simulink model "rc_sbus_encoder"  (R2026b)
settings: Solver=VariableStepAuto
undefined symbols (not defined in the file or in its folder): P, Ts
libraries: simulink x4
settings Model: Creator=aomar  LastModifiedBy=aomar

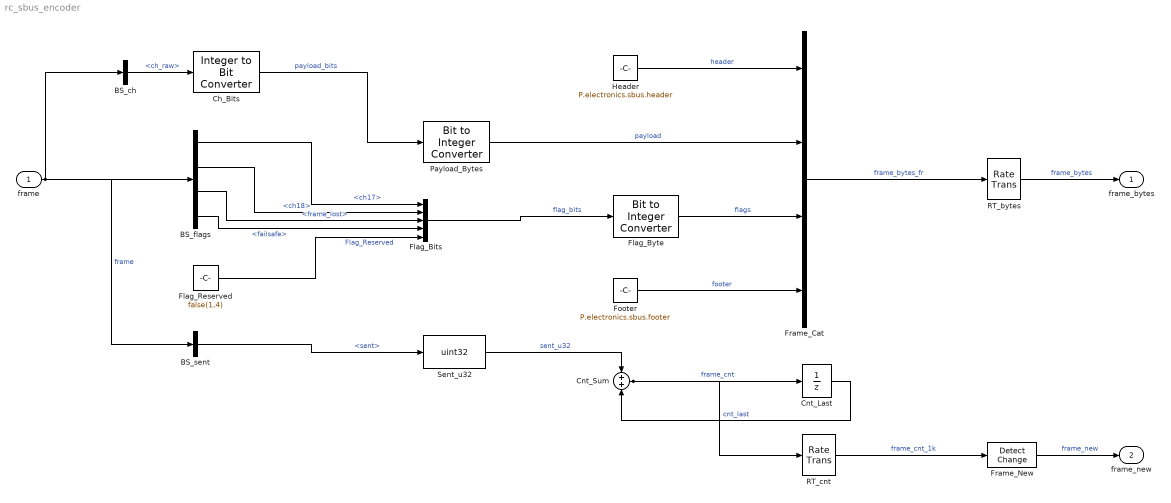
== system rc_sbus_encoder ==
  frame : Inport  OutDataTypeStr=Bus: Bus_RcFrame  SampleTime=Ts.rc_frame
  BS_ch : BusSelector  OutputSignals=ch_raw
  BS_flags : BusSelector  OutputSignals=ch17,ch18,frame_lost,failsafe
  BS_sent : BusSelector  OutputSignals=sent
  Ch_Bits : simulink/Logic and Bit Operations/Integer to Bit Converter  nbits=P.electronics.sbus.ch_bits  signedInputValues=Unsigned  bitOrder=LSB first  outDtype=boolean
      settings: LibrarySourceBlock=|
      | commutil2/Integer to Bit
      | Converter
  Cnt_Last : UnitDelay  SampleTime=Ts.rc_frame
  Cnt_Sum : Sum  OutDataTypeStr=uint32
  Flag_Bits : Concatenate  NumInputs=5
  Flag_Byte : simulink/Logic and Bit Operations/Bit to Integer Converter  nbits=8  bitOrder=LSB first  signedOutputValues=Unsigned  outDtype=uint8  outDtypeSigned=Inherit via internal rule
      settings: LibrarySourceBlock=|
      | commutil2/Bit to Integer
      | Converter
  Flag_Reserved : Constant  Value=false(1,4)  OutDataTypeStr=boolean  SampleTime=Ts.rc_frame
  Footer : Constant  Value=P.electronics.sbus.footer  OutDataTypeStr=uint8  SampleTime=Ts.rc_frame
  Frame_Cat : Concatenate  NumInputs=4
  Frame_New : simulink/Logic and Bit Operations/Detect Change  vinit=0  OutDataTypeStr=boolean
  Header : Constant  Value=P.electronics.sbus.header  OutDataTypeStr=uint8  SampleTime=Ts.rc_frame
  Payload_Bytes : simulink/Logic and Bit Operations/Bit to Integer Converter  nbits=8  bitOrder=LSB first  signedOutputValues=Unsigned  outDtype=uint8  outDtypeSigned=Inherit via internal rule
      settings: LibrarySourceBlock=|
      | commutil2/Bit to Integer
      | Converter
  RT_bytes : RateTransition  OutPortSampleTime=Ts.base
  RT_cnt : RateTransition  OutPortSampleTime=Ts.base
  Sent_u32 : DataTypeConversion  OutDataTypeStr=uint32  SaturateOnIntegerOverflow=off  RndMeth=Floor
  frame_bytes : Outport  OutDataTypeStr=uint8  PortDimensions=P.electronics.sbus.frame_len  SampleTime=Ts.base
  frame_new : Outport  Port=2  OutDataTypeStr=boolean  PortDimensions=1  SampleTime=Ts.base
  wires:
  frame/1 -> BS_sent/1, BS_ch/1, BS_flags/1  "frame"
  BS_ch/1 -> Ch_Bits/1  "<ch_raw>"
  BS_flags/1 -> Flag_Bits/1  "<ch17>"
  BS_flags/2 -> Flag_Bits/2  "<ch18>"
  BS_flags/3 -> Flag_Bits/3  "<frame_lost>"
  BS_flags/4 -> Flag_Bits/4  "<failsafe>"
  BS_sent/1 -> Sent_u32/1  "<sent>"
  Flag_Reserved/1 -> Flag_Bits/5  "Flag_Reserved"
  Ch_Bits/1 -> Payload_Bytes/1  "payload_bits"
  Flag_Bits/1 -> Flag_Byte/1  "flag_bits"
  Sent_u32/1 -> Cnt_Sum/1  "sent_u32"
  Payload_Bytes/1 -> Frame_Cat/2  "payload"
  Cnt_Sum/1 -> RT_cnt/1, Cnt_Last/1  "frame_cnt"
  Header/1 -> Frame_Cat/1  "header"
  Footer/1 -> Frame_Cat/4  "footer"
  Flag_Byte/1 -> Frame_Cat/3  "flags"
  Frame_Cat/1 -> RT_bytes/1  "frame_bytes_fr"
  Cnt_Last/1 -> Cnt_Sum/2  "cnt_last"
  RT_cnt/1 -> Frame_New/1  "frame_cnt_1k"
  RT_bytes/1 -> frame_bytes/1  "frame_bytes"
  Frame_New/1 -> frame_new/1  "frame_new"
